simulink model "BimanualCarvingModified"  (R2013a)
settings: Solver=ode4  SolverMode=SingleTasking  StartTime=0.0  StopTime=inf  FixedStep=0.0005  RelTol=1e-3
StartFcn:
  |  warndlg('Dexterit-E models cannot run under simulation. Please compile your model and run it from within Dexterit-E.');set_param(bdroot,'SimulationCommand','stop')
model workspace (MAT data in the model file):
  BKIN_STEP_TIME = 0.0005
  col_x = 1
  col_y = 2
  WIDTH = 3
  HEIGHT = 4
  TARGET_COL = 1
  LOAD = 2
  TRAJ_DURATION_COL = 3
  MAX_LOAD = 2
  FORCE_ON = 1
  HAND_RADIUS = 6
  REST_COL = 4
  TRAINING_COL = 5
  HAND_COLOR = 5
  TARGET_STROKE = 8
  TARGET_RADIUS = 9
  xMaxCursor = 15
  yMaxCursor = 16
  TARGET_COLOR = 7
  START_X = 10
  START_Y = 11
  STIFFNESS_MATERIAL = 3
  MATERIAL_MASS = 4
  MATERIAL_DAMPING = 5
  STIFFNESS_HANDS = 6
  MATERIAL_GOAL_COLOR = 12
  SCALE_VIBRATION = 7
  STONE_WIDTH = 6
  MATERIAL_DUCTILITY = 8
  TARG_COLOR = 1
  TEXT_COLOR = 13
  TEXTBOX_WIDTH = 14
  TEXTBOX_HEIGHT = 15
  ROTATION = 16
  LABEL_TEXT = 17
  LABEL_COLOR = 18
  LABEL_HEIGHT = 19
  ADVANCE_EMG_PLACEMENT = 2
  ADVANCE_EMG_MAX = 3
  EMG_ADVANCE_BUTTON = 1
  EMG_MVC_BUTTON = 2
  START_TRIAL = 3
  END_TRIAL = 4
  MUSC_NUM = 2
  HAND_DISTANCE = 3
  SYN_NUM = 4
  IS_R2_REAL = 5
  R2_SCORE_SD = 6
undefined symbols (not defined in the file or in its folder): slselsubs
libraries: xpclib x9, simulink x6, General x3, KINARM_loads x2, Video x2, KINARM_IO x1, KINARM_EP_loads x1
(part 2 of 6)

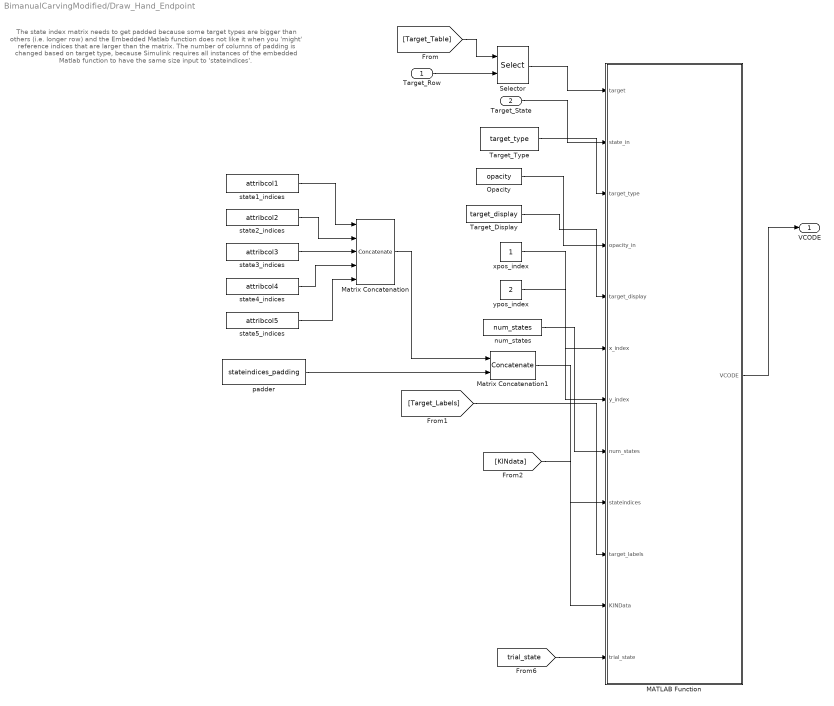
== system BimanualCarvingModified/Draw_Hand_Endpoint ==
  note: The state index matrix needs to get padded because
      | some target types are bigger than others (i.e. longer row)
      | and the Embedded Matlab function does not like it when you
      |  'might' reference indices that are larger than the matrix.
      |
      | The number of columns of padding is changed based on target
      | type, because Simulink requires all instances of the embedded
      | Matlab function to have the same size input to 'stateindices'.
  Target_Row : Inport
  Target_State : Inport  Port=2
  MATLAB Function : MATLAB Function  TreatAsAtomicUnit=on
  Matrix Concatenation : Concatenate  NumInputs=5  Mode=Multidimensional array
  Matrix Concatenation1 : Concatenate  Mode=Multidimensional array  ConcatenateDimension=2
  Opacity : Constant  Value=opacity
  Selector : Selector  NumberOfDimensions=2  InputPortWidth=3  IndexOptions=Index vector (port),Select all  Indices=1,-1  OutputSizes=slselsubs([(-2),(-2)],1),slselsubs([(-2),(-2)],2)
  Target_Display : Constant  Value=target_display
  Target_Type : Constant  Value=target_type
  num_states : Constant  Value=num_states
  padder : Constant  Value=stateindices_padding
  state1_indices : Constant  Value=attribcol1  VectorParams1D=off
  state2_indices : Constant  Value=attribcol2  VectorParams1D=off
  state3_indices : Constant  Value=attribcol3  VectorParams1D=off
  state4_indices : Constant  Value=attribcol4  VectorParams1D=off
  state5_indices : Constant  Value=attribcol5  VectorParams1D=off
  xpos_index : Constant
  ypos_index : Constant  Value=2
  VCODE : Outport  PortDimensions=[2 70]
  wires:
  Target_Display/1 -> MATLAB Function/5(target_display)
  state2_indices/1 -> Matrix Concatenation/2
  state1_indices/1 -> Matrix Concatenation/1
  [Target_Labels] -> MATLAB Function/10(target_labels)
  Target_Row/1 -> Selector/2
  [Target_Table] -> Selector/1
  Selector/1 -> MATLAB Function/1(target)
  Target_State/1 -> MATLAB Function/2(state_in)
  MATLAB Function/1(VCODE) -> VCODE/1
  xpos_index/1 -> MATLAB Function/6(x_index)
  ypos_index/1 -> MATLAB Function/7(y_index)
  num_states/1 -> MATLAB Function/8(num_states)
  Matrix Concatenation/1 -> Matrix Concatenation1/1
  padder/1 -> Matrix Concatenation1/2
  Matrix Concatenation1/1 -> MATLAB Function/9(stateindices)
  state3_indices/1 -> Matrix Concatenation/3
  state4_indices/1 -> Matrix Concatenation/4
  state5_indices/1 -> Matrix Concatenation/5
  Opacity/1 -> MATLAB Function/4(opacity_in)
  Target_Type/1 -> MATLAB Function/3(target_type)
  [KINdata] -> MATLAB Function/11(KINData)
  [trial_state] -> MATLAB Function/12(trial_state)

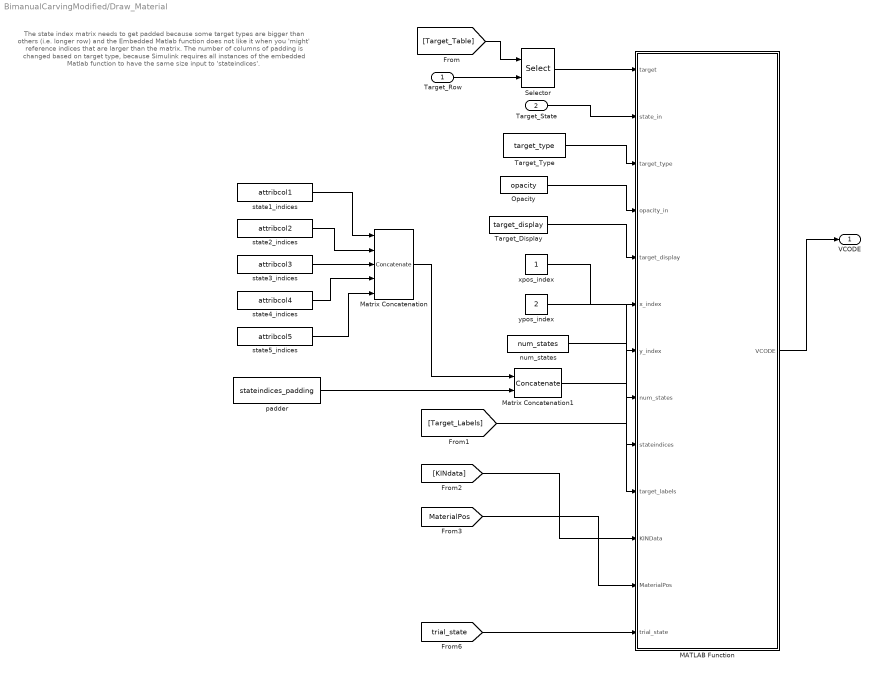
== system BimanualCarvingModified/Draw_Material ==
  note: The state index matrix needs to get padded because
      | some target types are bigger than others (i.e. longer row)
      | and the Embedded Matlab function does not like it when you
      |  'might' reference indices that are larger than the matrix.
      |
      | The number of columns of padding is changed based on target
      | type, because Simulink requires all instances of the embedded
      | Matlab function to have the same size input to 'stateindices'.
  Target_Row : Inport
  Target_State : Inport  Port=2
  MATLAB Function : MATLAB Function  TreatAsAtomicUnit=on
  Matrix Concatenation : Concatenate  NumInputs=5  Mode=Multidimensional array
  Matrix Concatenation1 : Concatenate  Mode=Multidimensional array  ConcatenateDimension=2
  Opacity : Constant  Value=opacity
  Selector : Selector  NumberOfDimensions=2  InputPortWidth=3  IndexOptions=Index vector (port),Select all  Indices=1,-1  OutputSizes=slselsubs([(-2),(-2)],1),slselsubs([(-2),(-2)],2)
  Target_Display : Constant  Value=target_display
  Target_Type : Constant  Value=target_type
  num_states : Constant  Value=num_states
  padder : Constant  Value=stateindices_padding
  state1_indices : Constant  Value=attribcol1  VectorParams1D=off
  state2_indices : Constant  Value=attribcol2  VectorParams1D=off
  state3_indices : Constant  Value=attribcol3  VectorParams1D=off
  state4_indices : Constant  Value=attribcol4  VectorParams1D=off
  state5_indices : Constant  Value=attribcol5  VectorParams1D=off
  xpos_index : Constant
  ypos_index : Constant  Value=2
  VCODE : Outport
  wires:
  Target_Display/1 -> MATLAB Function/5(target_display)
  state2_indices/1 -> Matrix Concatenation/2
  state1_indices/1 -> Matrix Concatenation/1
  [Target_Labels] -> MATLAB Function/10(target_labels)
  Target_Row/1 -> Selector/2
  [Target_Table] -> Selector/1
  Selector/1 -> MATLAB Function/1(target)
  Target_State/1 -> MATLAB Function/2(state_in)
  MATLAB Function/1(VCODE) -> VCODE/1
  xpos_index/1 -> MATLAB Function/6(x_index)
  ypos_index/1 -> MATLAB Function/7(y_index)
  num_states/1 -> MATLAB Function/8(num_states)
  Matrix Concatenation/1 -> Matrix Concatenation1/1
  padder/1 -> Matrix Concatenation1/2
  Matrix Concatenation1/1 -> MATLAB Function/9(stateindices)
  state3_indices/1 -> Matrix Concatenation/3
  state4_indices/1 -> Matrix Concatenation/4
  state5_indices/1 -> Matrix Concatenation/5
  Opacity/1 -> MATLAB Function/4(opacity_in)
  Target_Type/1 -> MATLAB Function/3(target_type)
  [KINdata] -> MATLAB Function/11(KINData)
  [MaterialPos] -> MATLAB Function/12(MaterialPos)
  [trial_state] -> MATLAB Function/13(trial_state)

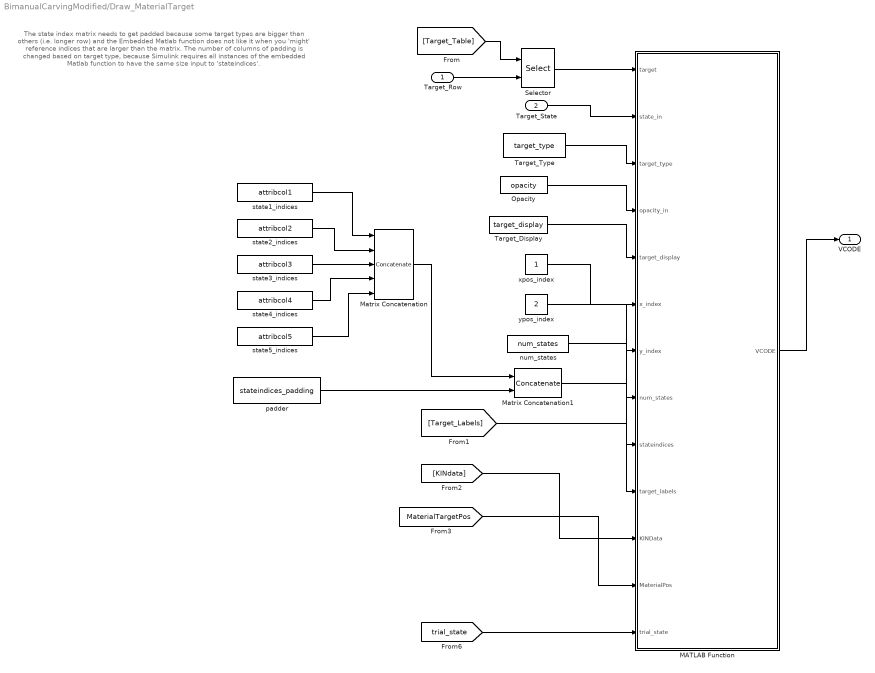
== system BimanualCarvingModified/Draw_MaterialTarget ==
  note: The state index matrix needs to get padded because
      | some target types are bigger than others (i.e. longer row)
      | and the Embedded Matlab function does not like it when you
      |  'might' reference indices that are larger than the matrix.
      |
      | The number of columns of padding is changed based on target
      | type, because Simulink requires all instances of the embedded
      | Matlab function to have the same size input to 'stateindices'.
  Target_Row : Inport
  Target_State : Inport  Port=2
  MATLAB Function : MATLAB Function  TreatAsAtomicUnit=on
  Matrix Concatenation : Concatenate  NumInputs=5  Mode=Multidimensional array
  Matrix Concatenation1 : Concatenate  Mode=Multidimensional array  ConcatenateDimension=2
  Opacity : Constant  Value=opacity
  Selector : Selector  NumberOfDimensions=2  InputPortWidth=3  IndexOptions=Index vector (port),Select all  Indices=1,-1  OutputSizes=slselsubs([(-2),(-2)],1),slselsubs([(-2),(-2)],2)
  Target_Display : Constant  Value=target_display
  Target_Type : Constant  Value=target_type
  num_states : Constant  Value=num_states
  padder : Constant  Value=stateindices_padding
  state1_indices : Constant  Value=attribcol1  VectorParams1D=off
  state2_indices : Constant  Value=attribcol2  VectorParams1D=off
  state3_indices : Constant  Value=attribcol3  VectorParams1D=off
  state4_indices : Constant  Value=attribcol4  VectorParams1D=off
  state5_indices : Constant  Value=attribcol5  VectorParams1D=off
  xpos_index : Constant
  ypos_index : Constant  Value=2
  VCODE : Outport
  wires:
  Target_Display/1 -> MATLAB Function/5(target_display)
  state2_indices/1 -> Matrix Concatenation/2
  state1_indices/1 -> Matrix Concatenation/1
  [Target_Labels] -> MATLAB Function/10(target_labels)
  Target_Row/1 -> Selector/2
  [Target_Table] -> Selector/1
  Selector/1 -> MATLAB Function/1(target)
  Target_State/1 -> MATLAB Function/2(state_in)
  MATLAB Function/1(VCODE) -> VCODE/1
  xpos_index/1 -> MATLAB Function/6(x_index)
  ypos_index/1 -> MATLAB Function/7(y_index)
  num_states/1 -> MATLAB Function/8(num_states)
  Matrix Concatenation/1 -> Matrix Concatenation1/1
  padder/1 -> Matrix Concatenation1/2
  Matrix Concatenation1/1 -> MATLAB Function/9(stateindices)
  state3_indices/1 -> Matrix Concatenation/3
  state4_indices/1 -> Matrix Concatenation/4
  state5_indices/1 -> Matrix Concatenation/5
  Opacity/1 -> MATLAB Function/4(opacity_in)
  Target_Type/1 -> MATLAB Function/3(target_type)
  [KINdata] -> MATLAB Function/11(KINData)
  [MaterialTargetPos] -> MATLAB Function/12(MaterialPos)
  [trial_state] -> MATLAB Function/13(trial_state)

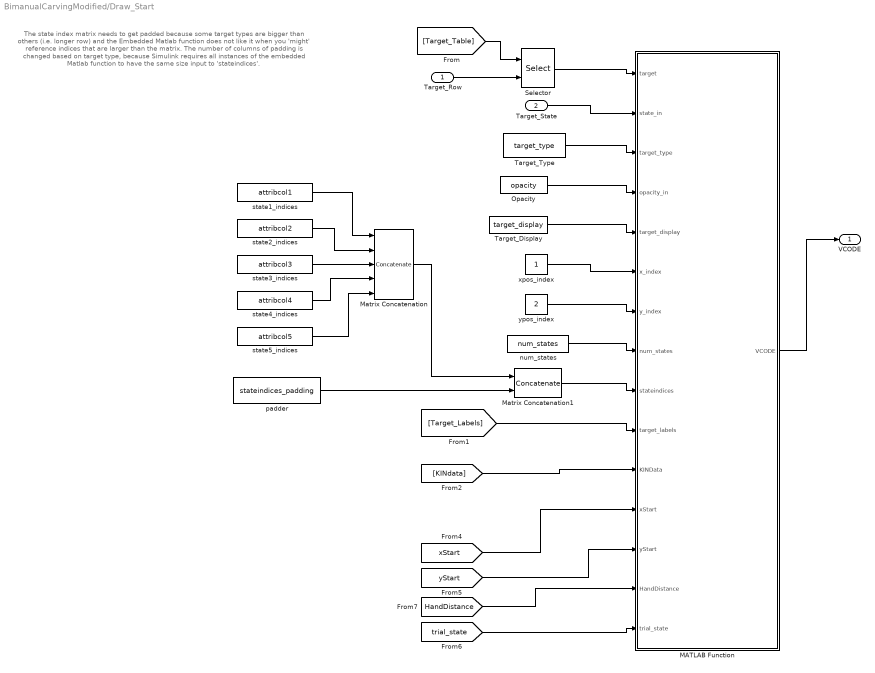
== system BimanualCarvingModified/Draw_Start ==
  note: The state index matrix needs to get padded because
      | some target types are bigger than others (i.e. longer row)
      | and the Embedded Matlab function does not like it when you
      |  'might' reference indices that are larger than the matrix.
      |
      | The number of columns of padding is changed based on target
      | type, because Simulink requires all instances of the embedded
      | Matlab function to have the same size input to 'stateindices'.
  Target_Row : Inport
  Target_State : Inport  Port=2
  MATLAB Function : MATLAB Function  TreatAsAtomicUnit=on
  Matrix Concatenation : Concatenate  NumInputs=5  Mode=Multidimensional array
  Matrix Concatenation1 : Concatenate  Mode=Multidimensional array  ConcatenateDimension=2
  Opacity : Constant  Value=opacity
  Selector : Selector  NumberOfDimensions=2  InputPortWidth=3  IndexOptions=Index vector (port),Select all  Indices=1,-1  OutputSizes=slselsubs([(-2),(-2)],1),slselsubs([(-2),(-2)],2)
  Target_Display : Constant  Value=target_display
  Target_Type : Constant  Value=target_type
  num_states : Constant  Value=num_states
  padder : Constant  Value=stateindices_padding
  state1_indices : Constant  Value=attribcol1  VectorParams1D=off
  state2_indices : Constant  Value=attribcol2  VectorParams1D=off
  state3_indices : Constant  Value=attribcol3  VectorParams1D=off
  state4_indices : Constant  Value=attribcol4  VectorParams1D=off
  state5_indices : Constant  Value=attribcol5  VectorParams1D=off
  xpos_index : Constant
  ypos_index : Constant  Value=2
  VCODE : Outport  PortDimensions=[2 70]
  wires:
  Target_Display/1 -> MATLAB Function/5(target_display)
  state2_indices/1 -> Matrix Concatenation/2
  state1_indices/1 -> Matrix Concatenation/1
  [Target_Labels] -> MATLAB Function/10(target_labels)
  Target_Row/1 -> Selector/2
  [Target_Table] -> Selector/1
  Selector/1 -> MATLAB Function/1(target)
  Target_State/1 -> MATLAB Function/2(state_in)
  MATLAB Function/1(VCODE) -> VCODE/1
  xpos_index/1 -> MATLAB Function/6(x_index)
  ypos_index/1 -> MATLAB Function/7(y_index)
  num_states/1 -> MATLAB Function/8(num_states)
  Matrix Concatenation/1 -> Matrix Concatenation1/1
  padder/1 -> Matrix Concatenation1/2
  Matrix Concatenation1/1 -> MATLAB Function/9(stateindices)
  state3_indices/1 -> Matrix Concatenation/3
  state4_indices/1 -> Matrix Concatenation/4
  state5_indices/1 -> Matrix Concatenation/5
  Opacity/1 -> MATLAB Function/4(opacity_in)
  Target_Type/1 -> MATLAB Function/3(target_type)
  [KINdata] -> MATLAB Function/11(KINData)
  [xStart] -> MATLAB Function/12(xStart)
  [trial_state] -> MATLAB Function/15(trial_state)
  [yStart] -> MATLAB Function/13(yStart)
  [HandDistance] -> MATLAB Function/14(HandDistance)

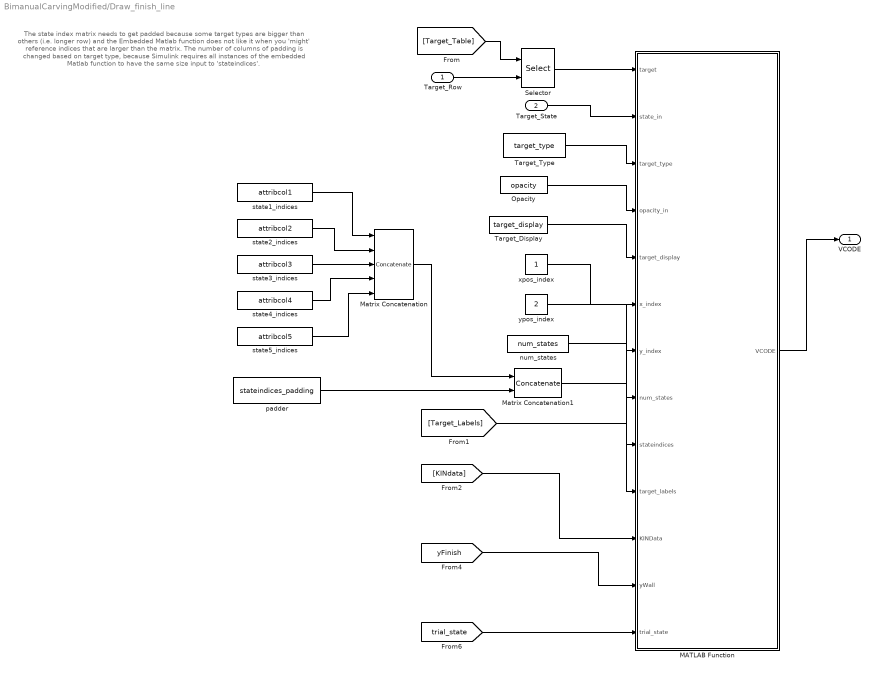
== system BimanualCarvingModified/Draw_finish_line ==
  note: The state index matrix needs to get padded because
      | some target types are bigger than others (i.e. longer row)
      | and the Embedded Matlab function does not like it when you
      |  'might' reference indices that are larger than the matrix.
      |
      | The number of columns of padding is changed based on target
      | type, because Simulink requires all instances of the embedded
      | Matlab function to have the same size input to 'stateindices'.
  Target_Row : Inport
  Target_State : Inport  Port=2
  MATLAB Function : MATLAB Function  TreatAsAtomicUnit=on
  Matrix Concatenation : Concatenate  NumInputs=5  Mode=Multidimensional array
  Matrix Concatenation1 : Concatenate  Mode=Multidimensional array  ConcatenateDimension=2
  Opacity : Constant  Value=opacity
  Selector : Selector  NumberOfDimensions=2  InputPortWidth=3  IndexOptions=Index vector (port),Select all  Indices=1,-1  OutputSizes=slselsubs([(-2),(-2)],1),slselsubs([(-2),(-2)],2)
  Target_Display : Constant  Value=target_display
  Target_Type : Constant  Value=target_type
  num_states : Constant  Value=num_states
  padder : Constant  Value=stateindices_padding
  state1_indices : Constant  Value=attribcol1  VectorParams1D=off
  state2_indices : Constant  Value=attribcol2  VectorParams1D=off
  state3_indices : Constant  Value=attribcol3  VectorParams1D=off
  state4_indices : Constant  Value=attribcol4  VectorParams1D=off
  state5_indices : Constant  Value=attribcol5  VectorParams1D=off
  xpos_index : Constant
  ypos_index : Constant  Value=2
  VCODE : Outport
  wires:
  Target_Display/1 -> MATLAB Function/5(target_display)
  state2_indices/1 -> Matrix Concatenation/2
  state1_indices/1 -> Matrix Concatenation/1
  [Target_Labels] -> MATLAB Function/10(target_labels)
  Target_Row/1 -> Selector/2
  [Target_Table] -> Selector/1
  Selector/1 -> MATLAB Function/1(target)
  Target_State/1 -> MATLAB Function/2(state_in)
  MATLAB Function/1(VCODE) -> VCODE/1
  xpos_index/1 -> MATLAB Function/6(x_index)
  ypos_index/1 -> MATLAB Function/7(y_index)
  num_states/1 -> MATLAB Function/8(num_states)
  Matrix Concatenation/1 -> Matrix Concatenation1/1
  padder/1 -> Matrix Concatenation1/2
  Matrix Concatenation1/1 -> MATLAB Function/9(stateindices)
  state3_indices/1 -> Matrix Concatenation/3
  state4_indices/1 -> Matrix Concatenation/4
  state5_indices/1 -> Matrix Concatenation/5
  Opacity/1 -> MATLAB Function/4(opacity_in)
  Target_Type/1 -> MATLAB Function/3(target_type)
  [KINdata] -> MATLAB Function/11(KINData)
  [yFinish] -> MATLAB Function/12(yWall)
  [trial_state] -> MATLAB Function/13(trial_state)

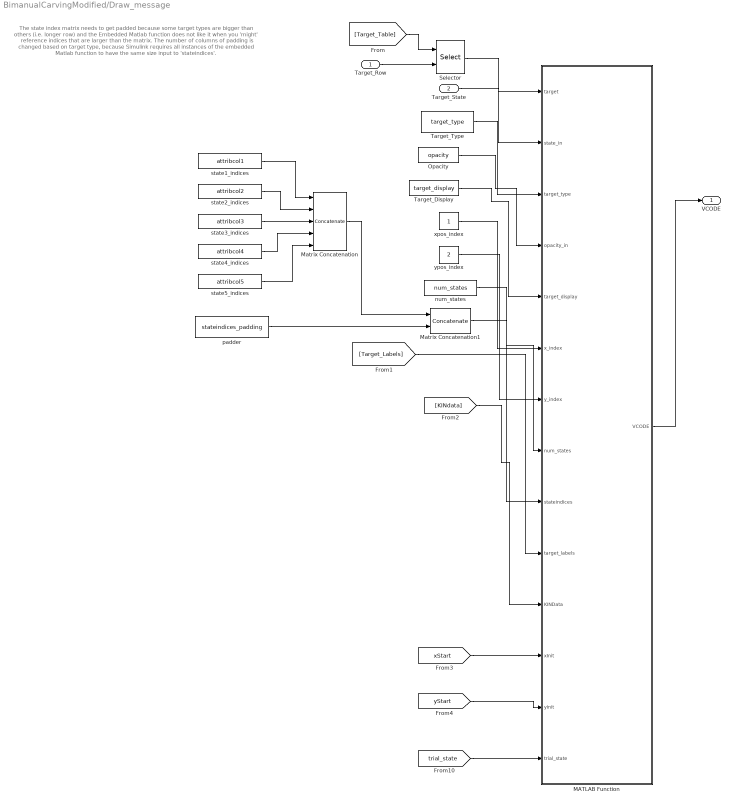
== system BimanualCarvingModified/Draw_message ==
  note: The state index matrix needs to get padded because
      | some target types are bigger than others (i.e. longer row)
      | and the Embedded Matlab function does not like it when you
      |  'might' reference indices that are larger than the matrix.
      |
      | The number of columns of padding is changed based on target
      | type, because Simulink requires all instances of the embedded
      | Matlab function to have the same size input to 'stateindices'.
  Target_Row : Inport
  Target_State : Inport  Port=2
  MATLAB Function : MATLAB Function  TreatAsAtomicUnit=on
  Matrix Concatenation : Concatenate  NumInputs=5  Mode=Multidimensional array
  Matrix Concatenation1 : Concatenate  Mode=Multidimensional array  ConcatenateDimension=2
  Opacity : Constant  Value=opacity
  Selector : Selector  NumberOfDimensions=2  InputPortWidth=3  IndexOptions=Index vector (port),Select all  Indices=1,-1  OutputSizes=slselsubs([(-2),(-2)],1),slselsubs([(-2),(-2)],2)
  Target_Display : Constant  Value=target_display
  Target_Type : Constant  Value=target_type
  num_states : Constant  Value=num_states
  padder : Constant  Value=stateindices_padding
  state1_indices : Constant  Value=attribcol1  VectorParams1D=off
  state2_indices : Constant  Value=attribcol2  VectorParams1D=off
  state3_indices : Constant  Value=attribcol3  VectorParams1D=off
  state4_indices : Constant  Value=attribcol4  VectorParams1D=off
  state5_indices : Constant  Value=attribcol5  VectorParams1D=off
  xpos_index : Constant
  ypos_index : Constant  Value=2
  VCODE : Outport  PortDimensions=[1 70]
  wires:
  Target_Display/1 -> MATLAB Function/5(target_display)
  state2_indices/1 -> Matrix Concatenation/2
  state1_indices/1 -> Matrix Concatenation/1
  [Target_Labels] -> MATLAB Function/10(target_labels)
  Target_Row/1 -> Selector/2
  [Target_Table] -> Selector/1
  Selector/1 -> MATLAB Function/1(target)
  Target_State/1 -> MATLAB Function/2(state_in)
  MATLAB Function/1(VCODE) -> VCODE/1
  xpos_index/1 -> MATLAB Function/6(x_index)
  ypos_index/1 -> MATLAB Function/7(y_index)
  num_states/1 -> MATLAB Function/8(num_states)
  Matrix Concatenation/1 -> Matrix Concatenation1/1
  padder/1 -> Matrix Concatenation1/2
  Matrix Concatenation1/1 -> MATLAB Function/9(stateindices)
  state3_indices/1 -> Matrix Concatenation/3
  state4_indices/1 -> Matrix Concatenation/4
  state5_indices/1 -> Matrix Concatenation/5
  Opacity/1 -> MATLAB Function/4(opacity_in)
  Target_Type/1 -> MATLAB Function/3(target_type)
  [KINdata] -> MATLAB Function/11(KINData)
  [trial_state] -> MATLAB Function/14(trial_state)
  [xStart] -> MATLAB Function/12(xInit)
  [yStart] -> MATLAB Function/13(yInit)

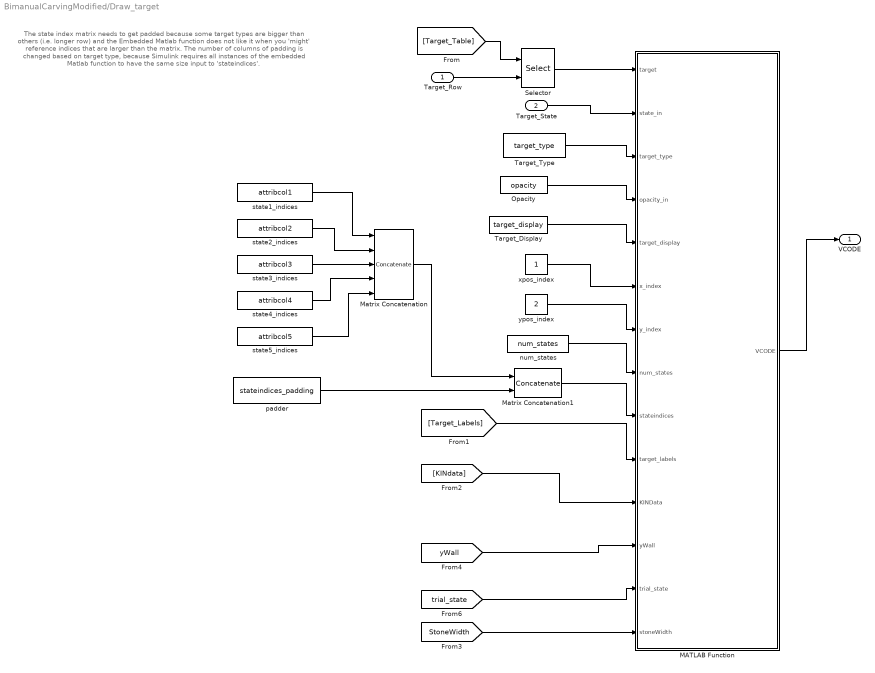
== system BimanualCarvingModified/Draw_target ==
  note: The state index matrix needs to get padded because
      | some target types are bigger than others (i.e. longer row)
      | and the Embedded Matlab function does not like it when you
      |  'might' reference indices that are larger than the matrix.
      |
      | The number of columns of padding is changed based on target
      | type, because Simulink requires all instances of the embedded
      | Matlab function to have the same size input to 'stateindices'.
  Target_Row : Inport
  Target_State : Inport  Port=2
  MATLAB Function : MATLAB Function  TreatAsAtomicUnit=on
  Matrix Concatenation : Concatenate  NumInputs=5  Mode=Multidimensional array
  Matrix Concatenation1 : Concatenate  Mode=Multidimensional array  ConcatenateDimension=2
  Opacity : Constant  Value=opacity
  Selector : Selector  NumberOfDimensions=2  InputPortWidth=3  IndexOptions=Index vector (port),Select all  Indices=1,-1  OutputSizes=slselsubs([(-2),(-2)],1),slselsubs([(-2),(-2)],2)
  Target_Display : Constant  Value=target_display
  Target_Type : Constant  Value=target_type
  num_states : Constant  Value=num_states
  padder : Constant  Value=stateindices_padding
  state1_indices : Constant  Value=attribcol1  VectorParams1D=off
  state2_indices : Constant  Value=attribcol2  VectorParams1D=off
  state3_indices : Constant  Value=attribcol3  VectorParams1D=off
  state4_indices : Constant  Value=attribcol4  VectorParams1D=off
  state5_indices : Constant  Value=attribcol5  VectorParams1D=off
  xpos_index : Constant
  ypos_index : Constant  Value=2
  VCODE : Outport
  wires:
  Target_Display/1 -> MATLAB Function/5(target_display)
  state2_indices/1 -> Matrix Concatenation/2
  state1_indices/1 -> Matrix Concatenation/1
  [Target_Labels] -> MATLAB Function/10(target_labels)
  Target_Row/1 -> Selector/2
  [Target_Table] -> Selector/1
  Selector/1 -> MATLAB Function/1(target)
  Target_State/1 -> MATLAB Function/2(state_in)
  MATLAB Function/1(VCODE) -> VCODE/1
  xpos_index/1 -> MATLAB Function/6(x_index)
  ypos_index/1 -> MATLAB Function/7(y_index)
  num_states/1 -> MATLAB Function/8(num_states)
  Matrix Concatenation/1 -> Matrix Concatenation1/1
  padder/1 -> Matrix Concatenation1/2
  Matrix Concatenation1/1 -> MATLAB Function/9(stateindices)
  state3_indices/1 -> Matrix Concatenation/3
  state4_indices/1 -> Matrix Concatenation/4
  state5_indices/1 -> Matrix Concatenation/5
  Opacity/1 -> MATLAB Function/4(opacity_in)
  Target_Type/1 -> MATLAB Function/3(target_type)
  [KINdata] -> MATLAB Function/11(KINData)
  [yWall] -> MATLAB Function/12(yWall)
  [trial_state] -> MATLAB Function/13(trial_state)
  [StoneWidth] -> MATLAB Function/14(stoneWidth)

== system BimanualCarvingModified/EMG Processing ==
  In1 : Inport
  In2 : Inport  Port=2
  In3 : Inport  Port=3
  In4 : Inport  Port=4
  Abs : Abs
  Filter : DiscreteFilter  Tag=BlockMethodSubSystem  Numerator=[6.1006178758066243e-05 0.00012201235751613249 6.1006178758066243e-05]  Denominator=[1 -1.9777864837767638 0.97803050849179607]  a0EqualsOne=on
  MATLAB Function1 : MATLAB Function  TreatAsAtomicUnit=on
  MATLAB Function2 : MATLAB Function  TreatAsAtomicUnit=on
  MATLAB Function3 : MATLAB Function  TreatAsAtomicUnit=on
  Out1 : Outport
  wires:
  Abs/1 -> Filter/1
  Filter/1 -> MATLAB Function1/1(emg), MATLAB Function3/1(emg), MATLAB Function2/1(emg)
  In3/1 -> MATLAB Function2/2(measure_max_emg)
  MATLAB Function2/1(maxemg) -> MATLAB Function3/2(max_emg)
  In4/1 -> MATLAB Function3/4(normalize)
  In2/1 -> MATLAB Function1/2(measure_min_emg)
  MATLAB Function3/1(output_emg) -> Out1/1
  In1/1 -> Abs/1
  MATLAB Function1/1(memg) -> MATLAB Function3/3(min_emg)

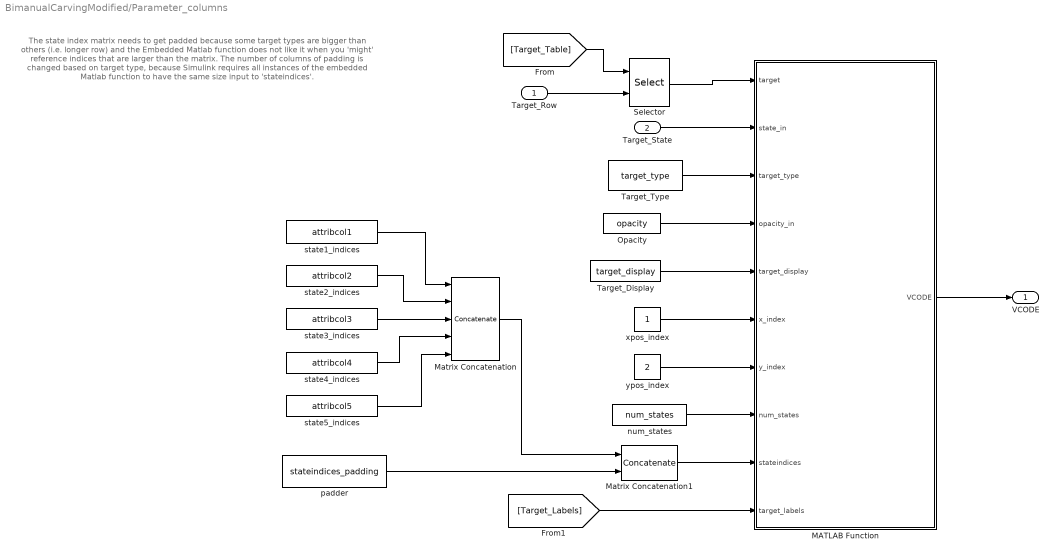
== system BimanualCarvingModified/Parameter_columns ==
  note: The state index matrix needs to get padded because
      | some target types are bigger than others (i.e. longer row)
      | and the Embedded Matlab function does not like it when you
      |  'might' reference indices that are larger than the matrix.
      |
      | The number of columns of padding is changed based on target
      | type, because Simulink requires all instances of the embedded
      | Matlab function to have the same size input to 'stateindices'.
  Target_Row : Inport
  Target_State : Inport  Port=2
  MATLAB Function : MATLAB Function  TreatAsAtomicUnit=on
  Matrix Concatenation : Concatenate  NumInputs=5  Mode=Multidimensional array
  Matrix Concatenation1 : Concatenate  Mode=Multidimensional array  ConcatenateDimension=2
  Opacity : Constant  Value=opacity
  Selector : Selector  NumberOfDimensions=2  InputPortWidth=3  IndexOptions=Index vector (port),Select all  Indices=1,-1  OutputSizes=slselsubs([(-2),(-2)],1),slselsubs([(-2),(-2)],2)
  Target_Display : Constant  Value=target_display
  Target_Type : Constant  Value=target_type
  num_states : Constant  Value=num_states
  padder : Constant  Value=stateindices_padding
  state1_indices : Constant  Value=attribcol1  VectorParams1D=off
  state2_indices : Constant  Value=attribcol2  VectorParams1D=off
  state3_indices : Constant  Value=attribcol3  VectorParams1D=off
  state4_indices : Constant  Value=attribcol4  VectorParams1D=off
  state5_indices : Constant  Value=attribcol5  VectorParams1D=off
  xpos_index : Constant
  ypos_index : Constant  Value=2
  VCODE : Outport  PortDimensions=[1 70]
  wires:
  Target_Display/1 -> MATLAB Function/5(target_display)
  state2_indices/1 -> Matrix Concatenation/2
  state1_indices/1 -> Matrix Concatenation/1
  [Target_Labels] -> MATLAB Function/10(target_labels)
  Target_Row/1 -> Selector/2
  [Target_Table] -> Selector/1
  Selector/1 -> MATLAB Function/1(target)
  Target_State/1 -> MATLAB Function/2(state_in)
  MATLAB Function/1(VCODE) -> VCODE/1
  xpos_index/1 -> MATLAB Function/6(x_index)
  ypos_index/1 -> MATLAB Function/7(y_index)
  num_states/1 -> MATLAB Function/8(num_states)
  Matrix Concatenation/1 -> Matrix Concatenation1/1
  padder/1 -> Matrix Concatenation1/2
  Matrix Concatenation1/1 -> MATLAB Function/9(stateindices)
  state3_indices/1 -> Matrix Concatenation/3
  state4_indices/1 -> Matrix Concatenation/4
  state5_indices/1 -> Matrix Concatenation/5
  Opacity/1 -> MATLAB Function/4(opacity_in)
  Target_Type/1 -> MATLAB Function/3(target_type)

== system BimanualCarvingModified/Trajectory subsystem ==
  note: In the Position Controller dialog, the "Time base of desired Position input signal" was set to 0.001.
      | This value is different from the Simulink sample-time of 0.0005 for that signal because the calculations
      | that create that signal in the Create_Trajectory block are based on 1 kHz. Please see the Help for
      | Position Controller block for more details.
  Duration : Inport
  target_position : Inport  Port=2
  Create_Trajectory : Subsystem
  KINARM_EP_Position_Controller : Subsystem  AncestorBlock=KINARM_EP_loads/KINARM_EP_Position_Controller  mask(KINARM_EP_Position_Controller){use_dom_hand=on, inertias_for_FF=KINARM End Point robot, gain_choice=Standard Movement, sample_time=0.001}
      mask prompts: use_dom_hand "Position control on dominant arm"; inertias_for_FF "Inertias to include for feed-forward control:"; gain_choice "Controller Performance"; sample_time "Time base of desired position input signal (-1 for inherited):"
      mask help:
      | <P>The KINARM_EP_Position_Controller block creates loads on the KINARM End-Point robot that implement position control of the hand using a feedforward model and feedback control.
      | <P>
      | The optional feedforward model uses estimates of KINARM End-Point robot inertia to create an estimate of required forces. A PD feedback controller is added to ensure optimal control.  The "Standard Movement" controller performance setting is optimized for reaching movements.  The "Step Response" setting is optimized for fast movements.
      | <P>
      | Desired position input is the (x, y) end-point position (i.e. handle).
      | <P>
      | <b>NOTE: it is critical to set the timebase of the desired position input signal correctly. Failure to do so will lead to robot instability, possibly damaging the KINARM robot and/or leading to subject injury.</b>
      mask init:
      | block_path = gcb;  % store block path, as gcb may change with block operations
      | 
      | %%% Handle background colours if link status changes.  
      | checkBackgroundColour(block_path, 'KINARM_EP_loads');
      | 
      | % Handle the inertias_for_FF setting: swap the 'inertia_option' inport with a constant block or 
      | % vice versa, if necessary, so that it matches the setting.
      | block_type = get_param([block_path '/inertia_option'], 'BlockType');
      | 
      | if (inertias_for_FF == 1) && ~strcmp(block_type, 'Inport') || ...  % if a change is required...
      |    (inertias_for_FF > 1) && strcmp(block_type, 'Inport')
      |     
      |     % ...delete the existing block, ...
      |     pos = get_param([block_path '/inertia_option'], 'Position');
      |     delete_line(block_path, 'inertia_option/1', 'FF_FB_Position_Controller/7');
      |     delete_block([block_path '/inertia_option']);
      |     
      |     % ...add an Inport or a 0-value Constant in place of the previous block (according to
      |     % the new setting), update the signal width flag, and then...
      |     if (inertias_for_FF == 1) && ~strcmp(block_type, 'Inport')
      |         add_block('built-in/Inport', [block_path '/inertia_option']);
      |      else
      |         add_block('built-in/Constant', [block_path '/inertia_option']);
      |         set_param([block_path '/inertia_option'], 'Value', 'inertias_for_FF - 2');
      |     end
      |     
      |     % ...connect the new block.
      |     set_param([block_path '/inertia_option'], 'Position', pos);
      |     add_line(block_path, 'inertia_option/1', 'FF_FB_Position_Controller/7');
      | end
      | 
      | 
      | 
      | % Set the sample rate of the desired_position input port based on the 
      | % sample rate from the mask
      | inports = find_system(block_path, 'LookUnderMasks', 'all', 'FollowLinks', 'on', 'SearchDepth', 1, 'BlockType', 'Inport');
      | set_param(inports{1}, 'SampleTime', get_param(gcb, 'sample_time') );
      | 
      | % Ensure the inports appear in a fixed order, and for each inport found add
      | % to the list of drawing commands a command to label it.
      | for i = 1:length(inports)
      |     inport_name = char(get_param(inports(i), 'Name'));
      |     
      |     if strcmp(inport_name, 'inertia_option')
      |         port = '3';
      | 	elseif strcmp(inport_name, 'desired_position')
      |         port = '1';
      |  	else
      | 		port = '2';
      | 		% do nothing
      | 	end
      |     
      |     set_param([block_path '/' inport_name], 'Port', port);
      | end
      mask Help:
      | Used to create loads for position control at the hand (i.e. finger-tip).
      | 
      | <H2>Library </H2>
      | KINARM_EP_loads (sub-library of Dexterit-E)
      | 
      | 
      | <H2>Description </H2>
      | The KINARM_EP_Position_Controller block creates loads on the KINARM End-Point robot that implement position control of the hand using a feedforward model and feedback control.
      | 
      | The optional feedforward model uses estimates of KINARM End-Point robot inertia to create an estimate of required forces. A PD feedback controller is added to ensure optimal control.  The "Standard Movement" controller performance setting is optimized for reaching movements.  The "Step Response" setting is optimized for fast movements.
      | <P>
      | <B>desired_xy_position: </B> this vector input is the desired position (i.e. attractor point) that the position controller acts on.  It should either be a [1x2] vector input or a VCODE.
      | The expected coordinate system and units for this input are the global coordinate system and meters.
      | <P>
      | <B>e_reset: </B> this scalar input resets the velocity and acceleration to zero for the feed-forward portion of the position controller model when e_reset transitions from 0 to 1.  This input should be used whenever the desired_xy_position input is being reset to a different position.
      | <P>
      | <B>inertia_option: </B> this optional scalar input defines which inertias to include for the feed-forward model.  Valid values are defined below.
      | <P>
      | <B>Forces: </B> this vector output is in a global Cartesian coordinate space as per all other KINARM End-Point load blocks.  It must be wired to the KINARM_EP_Apply_Loads block to actually apply the loads to the KINARM End-Point Robot.  This output may be added to other Force outputs from other KINARM End-Point load blocks to create a composite load.
      | <P>
      | 
      | <H2>Parameters and Dialog Box</H2>
      | <P>
      | <B>Position control on dominant arm:</B> indicates whether or not this position control is applied to the dominant arm (checked box) or non-dominant arm (unchecked box).
      | <P>
      | <B>Inertias to include for feed-forward control: </B> <BR>
      | Choices are: <BR>
      | (port)<BR>
      | 0 - None <BR>
      | 1 - KINARM End-Point robot  <BR>
      | <P>
      | If the (port) option is chosen, then an inport will be created allowing dynamic control of the inertia options.
      | The value wired to the inport will be mapped to the inertial choise using the values specified here (i.e. appropriate values are from 0-1).
      | Otherwise the option chosen will determine which inertias are included for the feed-forward control.
      | <P>
      | <B>Controller Performance: </B> <BR>
      | Choices are: <BR>
      | 1 - Standard Movement <BR>
      | 2 - Step Response  <BR>
      | <P>
      | The "Standard Movement" option is optimized for movements similar to normal reaching movements and provides high stiffness, but is underdamped.
      | There can be large overshoot following high accelerations/decellerations.
      | <P>
      | The "Step Response" option is optimized to minimize overshoot to less than ~10% for step responses, but at the cost of a reduction in controller stiffness.
      | <P>
      | NOTE: choice of Controller Performance option does not affect systems with secondary encoders - they are optimized for both conditions, providing higher stiffness and reasonable damping.
      | The controller for systems with secondary encoders provides less than ~10% overshoot for step responses.
      | <P>
      | 
      | <B>Time base of desired position input signal (-1 for inherited from sample time):</B> <BR>
      | Defines the time base used to calculate velocity and acceleration from the desired position input signal (-1 will inherit the time base from the sample time of the desired position input signal).
      | It is critical that this time base is set correctly.
      | The time base MUST be set to the time base used to create the desired input signal, WHICH MAY NOT BE THE SAME as the sample time of the desired input signal.
      | <B>Failure to set this time base correctly will lead to robot instability, possibly damaging the KINARM robot and/or leading to subject injury. </B>
      | <BR>
      | <I>Note: to determine the sample time of a signal, first update the model, then either select View --> Sample Time Legend or press Cntl + J.</I>
      | <P>
      | For example, a Stateflow chart that creates a desired position signal will, by default, use the model's sample time (e.g. 0.0005 s).
      | However, that Stateflow chart may use a time base that can be any multiple of the sample time (e.g. 0.001 s, 0.005 s, etc).
      | If a Stateflow chart was updating the desired position every 0.001 seconds, but the output sample time was 0.0005, then the position signal over time will look like:
      | <P>
      | [... x0, x0, x1, x1, x2, x2, x3, x3 ...].
      | <P>
      | A velocity calculated using 0.0005 time base will be:
      | <P>
      | [... 0, x1-x0, 0, x2-x1, 0, x3-x2, 0 ...] / 0.0005
      | <P>
      | (i.e. velocity will be 0 every other sample).
      | Whereas the true velocity in this example should be calculated using a 0.001 time base to create:
      | <P>
      |  [... x1-x0, x2-x1, x3-x2, ...] / 0.001.
      | 
      | <H2>Related Blocks </H2>
      | KINARM_EP_Apply_Loads, Virtual_Trajectory
      mask TypeOptions inertias_for_FF: (port) | None | KINARM End Point robot
      mask TypeOptions gain_choice: Standard Movement | Step Response
      mask Callback sample_time:
      | %ensure that sample time parameter is valid
      | sample_time_param = str2num( get_param(gcb, 'sample_time') );
      | model_step_size = str2num(get_param(bdroot, 'FixedStep'));
      | 
      | %default value:
      | sample_time = -1;
      | 
      | % if parameter value is numeric, sample_time_param will not be empty
      | if ~isempty(sample_time_param)
      | % 	round the sample time to an integer multiple of model step size, if possible
      | 	if ~isempty(model_step_size) && (model_step_size > 0)
      | 		sample_time = round( sample_time_param / model_step_size ) * model_step_size;
      | 	else
      | 		sample_time = sample_time_param;
      | 	end
      | 
      | 	% if input value is <=0, set it = -1 (inherited)
      | 	if (sample_time <= 0)
      | 		sample_time = -1;
      | 	end
      | end
      | 
      | set_param(gcb, 'sample_time', num2str(sample_time) );
  KINARM_Exo_Position_Controller : KINARM_loads/KINARM_Exo_Position_Controller  use_dom_hand=on  KINARM_Type=Human  inertias_for_FF=KINARM robot  angles_or_XY=End-point (global x/y)  sample_time=0.001
  calculate robot scaling : Subsystem
  EP forces : Outport
  EXO Torques : Outport  Port=2
  wires:
  Create_Trajectory/2(reset_controller) -> KINARM_EP_Position_Controller/2(e_reset), KINARM_Exo_Position_Controller/2
  Create_Trajectory/1(virtual_position) -> KINARM_EP_Position_Controller/1(desired_xy_position), KINARM_Exo_Position_Controller/1
  KINARM_EP_Position_Controller/1(Forces) -> EP forces/1
  KINARM_Exo_Position_Controller/1 -> EXO Torques/1
  target_position/1 -> Create_Trajectory/3(target_position)
  Duration/1 -> Create_Trajectory/1(nominal_duration)
  [e_start] -> Create_Trajectory/2(e_start)
  calculate robot scaling/1(scaling) -> Create_Trajectory/4(robot scaling)

== system BimanualCarvingModified/Trajectory subsystem/Create_Trajectory ==
  note: The Virtual_Trajectory block creates bell-shaped profile virtual trajectory.
      | The output is a time-varying (x,y) position ('virtual_position').
      |
      | The trajectory position starts at the current virtual_position output and ends at the target_position.
      | The trajectory is initiated with the e_start input and lasts for a duration specified by the duration input.
      |
      | To change the current virtual position to the reset_position input, a rising-edge event needs to be sent to the e_reset_vp input
      | (i.e. this can be useful for position control, with the Run_Status wired into the e_reset input).
      | If such an event occurs during a virtual trajectory, the trajectory is halted immediately.
  nominal_duration : Inport
  e_start : Inport  Port=2
  target_position : Inport  Port=3
  robot scaling : Inport  Port=4
  Detect Change : simulink/Logic and Bit Operations/Detect Change  vinit=0  InputProcessing=Inherited  OutDataTypeStr=uint8
  Terminator : Terminator
  Virtual_Trajectory : Subsystem
  get_arm_info : MATLAB Function  TreatAsAtomicUnit=on
  use dominant hand : Constant
  virtual_position : Outport
  reset_controller : Outport  Port=2
  wires:
  Virtual_Trajectory/1(virtual_position) -> virtual_position/1
  nominal_duration/1 -> Virtual_Trajectory/1(duration)
  e_start/1 -> Detect Change/1
  target_position/1 -> Virtual_Trajectory/2(target_position)
  Detect Change/1 -> Virtual_Trajectory/4(e_start)
  use dominant hand/1 -> get_arm_info/1(use_dom_hand)
  [KINdata] -> get_arm_info/2(kinarm_data)
  get_arm_info/1(position) -> Virtual_Trajectory/3(reset_position)
  Virtual_Trajectory/3(reset_controller) -> reset_controller/1
  get_arm_info/2(task_status) -> Virtual_Trajectory/5(task_status)
  get_arm_info/3(robot_enabled) -> Virtual_Trajectory/6(robot_enabled)
  [Run_Status] -> get_arm_info/3(run_status)
  Virtual_Trajectory/2(traj_status) -> Terminator/1
  robot scaling/1 -> get_arm_info/4(scaling)

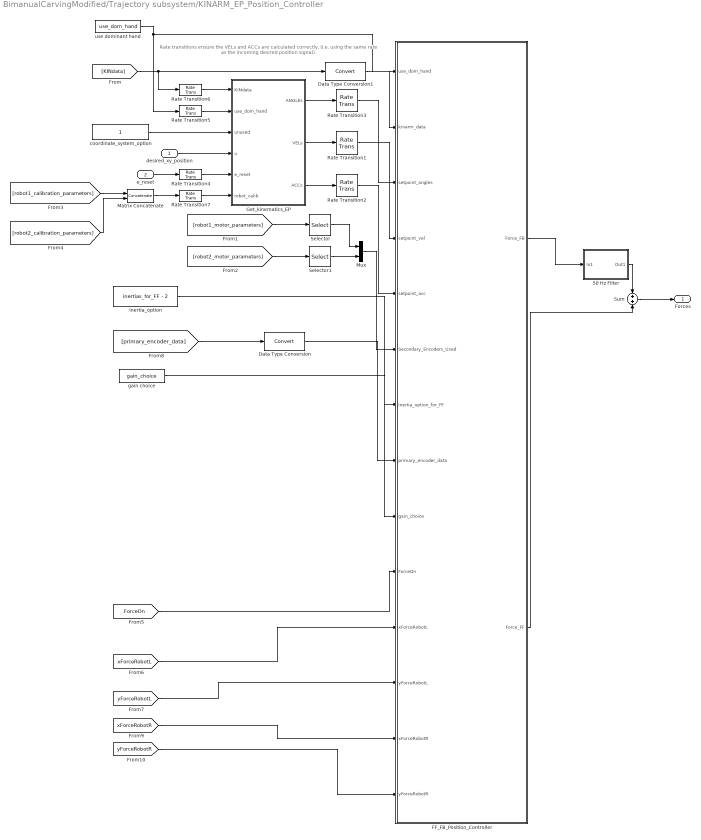
== system BimanualCarvingModified/Trajectory subsystem/KINARM_EP_Position_Controller ==
  note: Rate transitions ensure the VELs and ACCs are calculated correctly,
      | (i.e. using the same rate as the incoming desired position signal).
  desired_xy_position : Inport  SampleTime=0.001
  e_reset : Inport  Port=2
  50 Hz Filter : Subsystem
  Data Type Conversion : DataTypeConversion
  Data Type Conversion1 : DataTypeConversion
  FF_FB_Position_Controller : MATLAB Function  TreatAsAtomicUnit=on
  Get_kinematics_EP : Subsystem  SystemSampleTime=.001
  Matrix Concatenate : Concatenate  Mode=Multidimensional array  ConcatenateDimension=2
  Mux : Mux  Inputs=2
  Rate Transition{1..7} (7 alike) : RateTransition
  Selector : Selector  IndexOptions=Index vector (dialog)  Indices=6  OutputSizes=[(-2)]
  Selector1 : Selector  IndexOptions=Index vector (dialog)  Indices=6  OutputSizes=[(-2)]
  Sum : Sum
  coordinate_system_option : Constant
  gain choice : Constant  Value=gain_choice
  inertia_option : Constant  Value=inertias_for_FF - 2
  use dominant hand : Constant  Value=use_dom_hand
  Forces : Outport  SampleTime=[0 1]
  wires:
  Data Type Conversion1/1 -> FF_FB_Position_Controller/2(kinarm_data)
  desired_xy_position/1 -> Get_kinematics_EP/4(u)
  use dominant hand/1 -> FF_FB_Position_Controller/1(use_dom_hand), Rate Transition5/1
  [KINdata] -> Data Type Conversion1/1, Rate Transition6/1
  Sum/1 -> Forces/1
  FF_FB_Position_Controller/1(Force_FB) -> 50 Hz Filter/1(In1)
  FF_FB_Position_Controller/2(Force_FF) -> Sum/2
  50 Hz Filter/1(Out1) -> Sum/1
  Get_kinematics_EP/1(ANGLEs) -> Rate Transition3/1
  Get_kinematics_EP/2(VELs) -> Rate Transition1/1
  Get_kinematics_EP/3(ACCs) -> Rate Transition2/1
  e_reset/1 -> Rate Transition4/1
  [robot1_motor_parameters] -> Selector/1
  [robot2_motor_parameters] -> Selector1/1
  Selector/1 -> Mux/1
  Selector1/1 -> Mux/2
  Mux/1 -> FF_FB_Position_Controller/6(Secondary_Encoders_Used)
  [primary_encoder_data] -> Data Type Conversion/1
  Data Type Conversion/1 -> FF_FB_Position_Controller/8(primary_encoder_data)
  gain choice/1 -> FF_FB_Position_Controller/9(gain_choice)
  Rate Transition1/1 -> FF_FB_Position_Controller/4(setpoint_vel)
  Rate Transition2/1 -> FF_FB_Position_Controller/5(setpoint_acc)
  Rate Transition3/1 -> FF_FB_Position_Controller/3(setpoint_angles)
  Rate Transition4/1 -> Get_kinematics_EP/5(e_reset)
  Rate Transition5/1 -> Get_kinematics_EP/2(use_dom_hand)
  Rate Transition6/1 -> Get_kinematics_EP/1(KINdata)
  coordinate_system_option/1 -> Get_kinematics_EP/3(unused)
  Rate Transition7/1 -> Get_kinematics_EP/6(robot_calib)
  Matrix Concatenate/1 -> Rate Transition7/1
  [robot1_calibration_parameters] -> Matrix Concatenate/1
  [robot2_calibration_parameters] -> Matrix Concatenate/2
  inertia_option/1 -> FF_FB_Position_Controller/7(inertia_option_for_FF)
  [ForceOn] -> FF_FB_Position_Controller/10(ForceOn)
  [xForceRobotL] -> FF_FB_Position_Controller/11(xForceRobotL)
  [yForceRobotL] -> FF_FB_Position_Controller/12(yForceRobotL)
  [xForceRobotR] -> FF_FB_Position_Controller/13(xForceRobotR)
  [yForceRobotR] -> FF_FB_Position_Controller/14(yForceRobotR)

== system BimanualCarvingModified/Trajectory subsystem/calculate robot scaling ==
  MATLAB Function : MATLAB Function  TreatAsAtomicUnit=on
  Mux : Mux  Inputs=2
  Mux1 : Mux  Inputs=2
  Mux2 : Mux  Inputs=2
  Selector1 : Selector  InputPortWidth=9  IndexOptions=Index vector (dialog)  Indices=[7]  OutputSizes=[(-2)]
  Selector2 : Selector  InputPortWidth=9  IndexOptions=Index vector (dialog)  Indices=[7]  OutputSizes=[(-2)]
  scaling : Outport
  wires:
  [KINARMScalingRobot1] -> Mux/1
  [KINARMScalingRobot2] -> Mux/2
  Mux/1 -> MATLAB Function/2(exo_scaling)
  Mux1/1 -> MATLAB Function/3(ep_scaling)
  Mux2/1 -> MATLAB Function/1(robot_type)
  MATLAB Function/1(scaling) -> scaling/1
  [robot2_motor_parameters] -> Selector2/1
  Selector2/1 -> Mux2/2
  [KINARMEPScalingRobot2] -> Mux1/2
  [KINARMEPScalingRobot1] -> Mux1/1
  Selector1/1 -> Mux2/1
  [robot1_motor_parameters] -> Selector1/1
